simulink model "Horizontal1804"  (R2026b)
settings: Solver=FixedStepDiscrete  StopTime=inf  FixedStep=Official.Step
PostLoadFcn:
  | run(fullfile(fileparts(get_param('StampFly_IMU400','FileName')),'config','startup.m'));
InitFcn:
  | init_imu_flight;
undefined symbols (not defined in the file): Official
libraries: slpidlib x7, simulink x4, mspfiltlib x1
(part 4 of 5)

== system Horizontal1804/FlightControl/TakeoffHoverControl/AttitudeControl/RollAnglePID ==
  Error : Inport
  Dt : Inport  Port=2
  Reset : Inport  Port=3
  Enable : EnablePort
  DedicatedPID : slpidlib/PID Controller  Description=飛行比較用の専用PID。Ideal形式、台形積分・微分フィルター、実測Dt、単精度。  Controller=PID  Form=Ideal  TimeDomain=Discrete-time  UseExternalTs=on  SampleTime=.0025  IntegratorMethod=Trapezoidal  FilterMethod=Trapezoidal  ControllerParametersSource=internal  P=single(5)  I=single(1)/single(4)  UseKiTs=off  D=single(0.039999999105930328)  UseExternalDerivativeSource=off  N=single(1)/(single(0.125)*single(0.039999999105930328))  UseFilter=on  TunerSelectOption=Transfer Function Based (PID Tuner App)  InitialConditionSource=external  InitialConditionForIntegrator=0  InitialConditionForFilter=0  DifferentiatorICPrevScaledInput=0  ExternalReset=level  TrackingMode=off  Kt=1  LimitOutput=off  SatLimitsSource=internal  UpperSaturationLimit=inf  LowerSaturationLimit=-inf  LinearizeAsGain=off  AntiWindupMode=none  Kb=1  LimitIntegrator=on  UpperIntegratorSaturationLimit=single(30000)  LowerIntegratorSaturationLimit=single(-30000)  PGainOutDataTypeStr=single  PProdOutDataTypeStr=single  POutMin=[]  POutMax=[]  IGainOutDataTypeStr=single  IProdOutDataTypeStr=single  IOutMin=[]  IOutMax=[]  DGainOutDataTypeStr=single  DProdOutDataTypeStr=single  DOutMin=[]  DOutMax=[]  NGainOutDataTypeStr=single  NProdOutDataTypeStr=single  NOutMin=[]  NOutMax=[]  SumOutDataTypeStr=single  SumOutMin=[]  SumOutMax=[]  SaturationOutDataTypeStr=single  SaturationOutMin=[]  SaturationOutMax=[]  PParamDataTypeStr=single  PParamMin=[]  PParamMax=[]  IParamDataTypeStr=single  IParamMin=[]  IParamMax=[]  DParamDataTypeStr=single  DParamMin=[]  DParamMax=[]  NParamDataTypeStr=single  NParamMin=[]  NParamMax=[]  KbParamDataTypeStr=single  KbParamMin=[]  KbParamMax=[]  KtParamDataTypeStr=single  KtParamMin=[]  KtParamMax=[]  KbOutDataTypeStr=single  KbOutMin=[]  KbOutMax=[]  KtOutDataTypeStr=single  KtOutMin=[]  KtOutMax=[]  IntegratorOutDataTypeStr=single  IntegratorOutMin=[]  IntegratorOutMax=[]  FilterOutDataTypeStr=single  FilterOutMin=[]  FilterOutMax=[]  SumI1OutDataTypeStr=single  SumI1OutMin=[]  SumI1OutMax=[]  SumI2OutDataTypeStr=single  SumI2OutMin=[]  SumI2OutMax=[]  SumI3OutDataTypeStr=single  SumI3OutMin=[]  SumI3OutMax=[]  SumI4OutDataTypeStr=single  SumI4OutMin=[]  SumI4OutMax=[]  SumDOutDataTypeStr=single  SumDOutMin=[]  SumDOutMax=[]  SumAccumDataTypeStr=single  SumI1AccumDataTypeStr=single  SumI2AccumDataTypeStr=single  SumI3AccumDataTypeStr=single  SumI4AccumDataTypeStr=single  SumDAccumDataTypeStr=single  DifferentiatorOutDataTypeStr=single  DifferentiatorOutMin=[]  DifferentiatorOutMax=[]  FilterDiffOutCoefMin=[]  FilterDiffOutCoefMax=[]  ReciprocalOutDataTypeStr=single  ReciprocalOutMin=[]  ReciprocalOutMax=[]  SumDenOutDataTypeStr=single  SumDenOutMin=[]  SumDenOutMax=[]  SumNumOutDataTypeStr=single  SumNumOutMin=[]  SumNumOutMax=[]  SumDenAccumDataTypeStr=single  SumNumAccumDataTypeStr=single  DivideOutDataTypeStr=single  DivideOutMin=[]  DivideOutMax=[]  UdiffTsProdOutDataTypeStr=single  UdiffTsProdOutMin=[]  UdiffTsProdOutMax=[]  NTsProdOutDataTypeStr=single  NTsProdOutMin=[]  NTsProdOutMax=[]  UintegralTsProdOutDataTypeStr=single  UintegralTsProdOutMin=[]  UintegralTsProdOutMax=[]  UngainTsProdOutDataTypeStr=single  UngainTsProdOutMin=[]  UngainTsProdOutMax=[]  ClampingZeroOutDataTypeStr=single  ClampingZeroOutMin=[]  ClampingZeroOutMax=[]  FilterDenConstantOutDataTypeStr=single  FilterDenConstantOutMin=[]  FilterDenConstantOutMax=[]  PCopyOutDataTypeStr=single  PCopyOutMin=[]  PCopyOutMax=[]  NCopyOutDataTypeStr=single  NCopyOutMin=[]  NCopyOutMax=[]  IntegratorContinuousStateAttributes=''  IntegratorStateMustResolveToSignalObject=off  IntegratorRTWStateStorageClass=Auto  FilterContinuousStateAttributes=''  FilterStateMustResolveToSignalObject=off  FilterRTWStateStorageClass=Auto  ParallelPVariant=Passthrough  IdealPVariant=InternalParameters  IVariant=InternalParameters  DVariant=InternalParameters  IntegratorVariant=Discrete  SatVariant=Disabled  AWVariant=Passthrough  PCopyVariant=Disabled  TRVariant=Disabled  FdbkBlocksVariant=Forward  IdealPFdbkVariant=Disabled  SatFdbkVariant=Disabled  DerivativeFilterVariant=TrapezoidalFilter  NVariant=InternalParameters  NCopyVariant=InternalParameters  FilterICVariant=ExternalICs  IntegratorICVariant=ExternalICs  ExternalResetVariant=ExternalReset  TRSumVariant=Passthrough  SumFdbkVariant=Disabled  SumVariant=Sum_PID  TsampFilterVariant=ExternalTs  TsampNgainVariant=Passthrough  TsampIntegralVariant=ExternalTs  ExternalSaturationOutDataTypeStr=Inherit: Same as second input  DerivativeSourceVariant=ErrorSignal  PreIntVariant=InternalPreInt
      settings: LibrarySourceBlock=simulink/Discrete/Discrete PID Controller
  ZeroInitialCondition : Constant  Description=ZeroInitialCondition：固定値 single(0) を出力します。意味と単位は親の機能説明と信号名を参照します。  Value=single(0)
  Output : Outport
  wires:
  DedicatedPID/1 -> Output/1
  Dt/1 -> DedicatedPID/5
  ZeroInitialCondition/1 -> DedicatedPID/4, DedicatedPID/3
  Reset/1 -> DedicatedPID/2
  Error/1 -> DedicatedPID/1

== system Horizontal1804/FlightControl/TakeoffHoverControl/BodyRateControl/PitchRatePID ==
  Error : Inport
  Dt : Inport  Port=2
  Reset : Inport  Port=3
  Enable : EnablePort
  DedicatedPID : slpidlib/PID Controller  Description=飛行比較用の専用PID。Ideal形式、台形積分・微分フィルター、実測Dt、単精度。  Controller=PID  Form=Ideal  TimeDomain=Discrete-time  UseExternalTs=on  SampleTime=.0025  IntegratorMethod=Trapezoidal  FilterMethod=Trapezoidal  ControllerParametersSource=internal  P=single(0.94999998807907104)  I=single(1)/single(0.69999998807907104)  UseKiTs=off  D=single(0.02500000037252903)  UseExternalDerivativeSource=off  N=single(1)/(single(0.125)*single(0.02500000037252903))  UseFilter=on  TunerSelectOption=Transfer Function Based (PID Tuner App)  InitialConditionSource=external  InitialConditionForIntegrator=0  InitialConditionForFilter=0  DifferentiatorICPrevScaledInput=0  ExternalReset=level  TrackingMode=off  Kt=1  LimitOutput=off  SatLimitsSource=internal  UpperSaturationLimit=inf  LowerSaturationLimit=-inf  LinearizeAsGain=off  AntiWindupMode=none  Kb=1  LimitIntegrator=on  UpperIntegratorSaturationLimit=single(30000)  LowerIntegratorSaturationLimit=single(-30000)  PGainOutDataTypeStr=single  PProdOutDataTypeStr=single  POutMin=[]  POutMax=[]  IGainOutDataTypeStr=single  IProdOutDataTypeStr=single  IOutMin=[]  IOutMax=[]  DGainOutDataTypeStr=single  DProdOutDataTypeStr=single  DOutMin=[]  DOutMax=[]  NGainOutDataTypeStr=single  NProdOutDataTypeStr=single  NOutMin=[]  NOutMax=[]  SumOutDataTypeStr=single  SumOutMin=[]  SumOutMax=[]  SaturationOutDataTypeStr=single  SaturationOutMin=[]  SaturationOutMax=[]  PParamDataTypeStr=single  PParamMin=[]  PParamMax=[]  IParamDataTypeStr=single  IParamMin=[]  IParamMax=[]  DParamDataTypeStr=single  DParamMin=[]  DParamMax=[]  NParamDataTypeStr=single  NParamMin=[]  NParamMax=[]  KbParamDataTypeStr=single  KbParamMin=[]  KbParamMax=[]  KtParamDataTypeStr=single  KtParamMin=[]  KtParamMax=[]  KbOutDataTypeStr=single  KbOutMin=[]  KbOutMax=[]  KtOutDataTypeStr=single  KtOutMin=[]  KtOutMax=[]  IntegratorOutDataTypeStr=single  IntegratorOutMin=[]  IntegratorOutMax=[]  FilterOutDataTypeStr=single  FilterOutMin=[]  FilterOutMax=[]  SumI1OutDataTypeStr=single  SumI1OutMin=[]  SumI1OutMax=[]  SumI2OutDataTypeStr=single  SumI2OutMin=[]  SumI2OutMax=[]  SumI3OutDataTypeStr=single  SumI3OutMin=[]  SumI3OutMax=[]  SumI4OutDataTypeStr=single  SumI4OutMin=[]  SumI4OutMax=[]  SumDOutDataTypeStr=single  SumDOutMin=[]  SumDOutMax=[]  SumAccumDataTypeStr=single  SumI1AccumDataTypeStr=single  SumI2AccumDataTypeStr=single  SumI3AccumDataTypeStr=single  SumI4AccumDataTypeStr=single  SumDAccumDataTypeStr=single  DifferentiatorOutDataTypeStr=single  DifferentiatorOutMin=[]  DifferentiatorOutMax=[]  FilterDiffOutCoefMin=[]  FilterDiffOutCoefMax=[]  ReciprocalOutDataTypeStr=single  ReciprocalOutMin=[]  ReciprocalOutMax=[]  SumDenOutDataTypeStr=single  SumDenOutMin=[]  SumDenOutMax=[]  SumNumOutDataTypeStr=single  SumNumOutMin=[]  SumNumOutMax=[]  SumDenAccumDataTypeStr=single  SumNumAccumDataTypeStr=single  DivideOutDataTypeStr=single  DivideOutMin=[]  DivideOutMax=[]  UdiffTsProdOutDataTypeStr=single  UdiffTsProdOutMin=[]  UdiffTsProdOutMax=[]  NTsProdOutDataTypeStr=single  NTsProdOutMin=[]  NTsProdOutMax=[]  UintegralTsProdOutDataTypeStr=single  UintegralTsProdOutMin=[]  UintegralTsProdOutMax=[]  UngainTsProdOutDataTypeStr=single  UngainTsProdOutMin=[]  UngainTsProdOutMax=[]  ClampingZeroOutDataTypeStr=single  ClampingZeroOutMin=[]  ClampingZeroOutMax=[]  FilterDenConstantOutDataTypeStr=single  FilterDenConstantOutMin=[]  FilterDenConstantOutMax=[]  PCopyOutDataTypeStr=single  PCopyOutMin=[]  PCopyOutMax=[]  NCopyOutDataTypeStr=single  NCopyOutMin=[]  NCopyOutMax=[]  IntegratorContinuousStateAttributes=''  IntegratorStateMustResolveToSignalObject=off  IntegratorRTWStateStorageClass=Auto  FilterContinuousStateAttributes=''  FilterStateMustResolveToSignalObject=off  FilterRTWStateStorageClass=Auto  ParallelPVariant=Passthrough  IdealPVariant=InternalParameters  IVariant=InternalParameters  DVariant=InternalParameters  IntegratorVariant=Discrete  SatVariant=Disabled  AWVariant=Passthrough  PCopyVariant=Disabled  TRVariant=Disabled  FdbkBlocksVariant=Forward  IdealPFdbkVariant=Disabled  SatFdbkVariant=Disabled  DerivativeFilterVariant=TrapezoidalFilter  NVariant=InternalParameters  NCopyVariant=InternalParameters  FilterICVariant=ExternalICs  IntegratorICVariant=ExternalICs  ExternalResetVariant=ExternalReset  TRSumVariant=Passthrough  SumFdbkVariant=Disabled  SumVariant=Sum_PID  TsampFilterVariant=ExternalTs  TsampNgainVariant=Passthrough  TsampIntegralVariant=ExternalTs  ExternalSaturationOutDataTypeStr=Inherit: Same as second input  DerivativeSourceVariant=ErrorSignal  PreIntVariant=InternalPreInt
      settings: LibrarySourceBlock=simulink/Discrete/Discrete PID Controller
  ZeroInitialCondition : Constant  Description=ZeroInitialCondition：固定値 single(0) を出力します。意味と単位は親の機能説明と信号名を参照します。  Value=single(0)
  Output : Outport
  wires:
  DedicatedPID/1 -> Output/1
  Dt/1 -> DedicatedPID/5
  ZeroInitialCondition/1 -> DedicatedPID/4, DedicatedPID/3
  Reset/1 -> DedicatedPID/2
  Error/1 -> DedicatedPID/1

== system Horizontal1804/FlightControl/TakeoffHoverControl/BodyRateControl/RollRatePID ==
  Error : Inport
  Dt : Inport  Port=2
  Reset : Inport  Port=3
  Enable : EnablePort
  DedicatedPID : slpidlib/PID Controller  Description=飛行比較用の専用PID。Ideal形式、台形積分・微分フィルター、実測Dt、単精度。  Controller=PID  Form=Ideal  TimeDomain=Discrete-time  UseExternalTs=on  SampleTime=.0025  IntegratorMethod=Trapezoidal  FilterMethod=Trapezoidal  ControllerParametersSource=internal  P=single(0.64999997615814209)  I=single(1)/single(0.69999998807907104)  UseKiTs=off  D=single(0.0099999997764825821)  UseExternalDerivativeSource=off  N=single(1)/(single(0.125)*single(0.0099999997764825821))  UseFilter=on  TunerSelectOption=Transfer Function Based (PID Tuner App)  InitialConditionSource=external  InitialConditionForIntegrator=0  InitialConditionForFilter=0  DifferentiatorICPrevScaledInput=0  ExternalReset=level  TrackingMode=off  Kt=1  LimitOutput=off  SatLimitsSource=internal  UpperSaturationLimit=inf  LowerSaturationLimit=-inf  LinearizeAsGain=off  AntiWindupMode=none  Kb=1  LimitIntegrator=on  UpperIntegratorSaturationLimit=single(30000)  LowerIntegratorSaturationLimit=single(-30000)  PGainOutDataTypeStr=single  PProdOutDataTypeStr=single  POutMin=[]  POutMax=[]  IGainOutDataTypeStr=single  IProdOutDataTypeStr=single  IOutMin=[]  IOutMax=[]  DGainOutDataTypeStr=single  DProdOutDataTypeStr=single  DOutMin=[]  DOutMax=[]  NGainOutDataTypeStr=single  NProdOutDataTypeStr=single  NOutMin=[]  NOutMax=[]  SumOutDataTypeStr=single  SumOutMin=[]  SumOutMax=[]  SaturationOutDataTypeStr=single  SaturationOutMin=[]  SaturationOutMax=[]  PParamDataTypeStr=single  PParamMin=[]  PParamMax=[]  IParamDataTypeStr=single  IParamMin=[]  IParamMax=[]  DParamDataTypeStr=single  DParamMin=[]  DParamMax=[]  NParamDataTypeStr=single  NParamMin=[]  NParamMax=[]  KbParamDataTypeStr=single  KbParamMin=[]  KbParamMax=[]  KtParamDataTypeStr=single  KtParamMin=[]  KtParamMax=[]  KbOutDataTypeStr=single  KbOutMin=[]  KbOutMax=[]  KtOutDataTypeStr=single  KtOutMin=[]  KtOutMax=[]  IntegratorOutDataTypeStr=single  IntegratorOutMin=[]  IntegratorOutMax=[]  FilterOutDataTypeStr=single  FilterOutMin=[]  FilterOutMax=[]  SumI1OutDataTypeStr=single  SumI1OutMin=[]  SumI1OutMax=[]  SumI2OutDataTypeStr=single  SumI2OutMin=[]  SumI2OutMax=[]  SumI3OutDataTypeStr=single  SumI3OutMin=[]  SumI3OutMax=[]  SumI4OutDataTypeStr=single  SumI4OutMin=[]  SumI4OutMax=[]  SumDOutDataTypeStr=single  SumDOutMin=[]  SumDOutMax=[]  SumAccumDataTypeStr=single  SumI1AccumDataTypeStr=single  SumI2AccumDataTypeStr=single  SumI3AccumDataTypeStr=single  SumI4AccumDataTypeStr=single  SumDAccumDataTypeStr=single  DifferentiatorOutDataTypeStr=single  DifferentiatorOutMin=[]  DifferentiatorOutMax=[]  FilterDiffOutCoefMin=[]  FilterDiffOutCoefMax=[]  ReciprocalOutDataTypeStr=single  ReciprocalOutMin=[]  ReciprocalOutMax=[]  SumDenOutDataTypeStr=single  SumDenOutMin=[]  SumDenOutMax=[]  SumNumOutDataTypeStr=single  SumNumOutMin=[]  SumNumOutMax=[]  SumDenAccumDataTypeStr=single  SumNumAccumDataTypeStr=single  DivideOutDataTypeStr=single  DivideOutMin=[]  DivideOutMax=[]  UdiffTsProdOutDataTypeStr=single  UdiffTsProdOutMin=[]  UdiffTsProdOutMax=[]  NTsProdOutDataTypeStr=single  NTsProdOutMin=[]  NTsProdOutMax=[]  UintegralTsProdOutDataTypeStr=single  UintegralTsProdOutMin=[]  UintegralTsProdOutMax=[]  UngainTsProdOutDataTypeStr=single  UngainTsProdOutMin=[]  UngainTsProdOutMax=[]  ClampingZeroOutDataTypeStr=single  ClampingZeroOutMin=[]  ClampingZeroOutMax=[]  FilterDenConstantOutDataTypeStr=single  FilterDenConstantOutMin=[]  FilterDenConstantOutMax=[]  PCopyOutDataTypeStr=single  PCopyOutMin=[]  PCopyOutMax=[]  NCopyOutDataTypeStr=single  NCopyOutMin=[]  NCopyOutMax=[]  IntegratorContinuousStateAttributes=''  IntegratorStateMustResolveToSignalObject=off  IntegratorRTWStateStorageClass=Auto  FilterContinuousStateAttributes=''  FilterStateMustResolveToSignalObject=off  FilterRTWStateStorageClass=Auto  ParallelPVariant=Passthrough  IdealPVariant=InternalParameters  IVariant=InternalParameters  DVariant=InternalParameters  IntegratorVariant=Discrete  SatVariant=Disabled  AWVariant=Passthrough  PCopyVariant=Disabled  TRVariant=Disabled  FdbkBlocksVariant=Forward  IdealPFdbkVariant=Disabled  SatFdbkVariant=Disabled  DerivativeFilterVariant=TrapezoidalFilter  NVariant=InternalParameters  NCopyVariant=InternalParameters  FilterICVariant=ExternalICs  IntegratorICVariant=ExternalICs  ExternalResetVariant=ExternalReset  TRSumVariant=Passthrough  SumFdbkVariant=Disabled  SumVariant=Sum_PID  TsampFilterVariant=ExternalTs  TsampNgainVariant=Passthrough  TsampIntegralVariant=ExternalTs  ExternalSaturationOutDataTypeStr=Inherit: Same as second input  DerivativeSourceVariant=ErrorSignal  PreIntVariant=InternalPreInt
      settings: LibrarySourceBlock=simulink/Discrete/Discrete PID Controller
  ZeroInitialCondition : Constant  Description=ZeroInitialCondition：固定値 single(0) を出力します。意味と単位は親の機能説明と信号名を参照します。  Value=single(0)
  Output : Outport
  wires:
  DedicatedPID/1 -> Output/1
  Dt/1 -> DedicatedPID/5
  ZeroInitialCondition/1 -> DedicatedPID/3, DedicatedPID/4
  Reset/1 -> DedicatedPID/2
  Error/1 -> DedicatedPID/1

== system Horizontal1804/FlightControl/TakeoffHoverControl/BodyRateControl/YawRatePID ==
  Error : Inport
  Dt : Inport  Port=2
  Reset : Inport  Port=3
  Enable : EnablePort
  DedicatedPID : slpidlib/PID Controller  Description=飛行比較用の専用PID。Ideal形式、台形積分・微分フィルター、実測Dt、単精度。  Controller=PID  Form=Ideal  TimeDomain=Discrete-time  UseExternalTs=on  SampleTime=.0025  IntegratorMethod=Trapezoidal  FilterMethod=Trapezoidal  ControllerParametersSource=internal  P=single(3)  I=single(1)/single(0.80000001192092896)  UseKiTs=off  D=single(0.0099999997764825821)  UseExternalDerivativeSource=off  N=single(1)/(single(0.125)*single(0.0099999997764825821))  UseFilter=on  TunerSelectOption=Transfer Function Based (PID Tuner App)  InitialConditionSource=external  InitialConditionForIntegrator=0  InitialConditionForFilter=0  DifferentiatorICPrevScaledInput=0  ExternalReset=level  TrackingMode=off  Kt=1  LimitOutput=off  SatLimitsSource=internal  UpperSaturationLimit=inf  LowerSaturationLimit=-inf  LinearizeAsGain=off  AntiWindupMode=none  Kb=1  LimitIntegrator=on  UpperIntegratorSaturationLimit=single(30000)  LowerIntegratorSaturationLimit=single(-30000)  PGainOutDataTypeStr=single  PProdOutDataTypeStr=single  POutMin=[]  POutMax=[]  IGainOutDataTypeStr=single  IProdOutDataTypeStr=single  IOutMin=[]  IOutMax=[]  DGainOutDataTypeStr=single  DProdOutDataTypeStr=single  DOutMin=[]  DOutMax=[]  NGainOutDataTypeStr=single  NProdOutDataTypeStr=single  NOutMin=[]  NOutMax=[]  SumOutDataTypeStr=single  SumOutMin=[]  SumOutMax=[]  SaturationOutDataTypeStr=single  SaturationOutMin=[]  SaturationOutMax=[]  PParamDataTypeStr=single  PParamMin=[]  PParamMax=[]  IParamDataTypeStr=single  IParamMin=[]  IParamMax=[]  DParamDataTypeStr=single  DParamMin=[]  DParamMax=[]  NParamDataTypeStr=single  NParamMin=[]  NParamMax=[]  KbParamDataTypeStr=single  KbParamMin=[]  KbParamMax=[]  KtParamDataTypeStr=single  KtParamMin=[]  KtParamMax=[]  KbOutDataTypeStr=single  KbOutMin=[]  KbOutMax=[]  KtOutDataTypeStr=single  KtOutMin=[]  KtOutMax=[]  IntegratorOutDataTypeStr=single  IntegratorOutMin=[]  IntegratorOutMax=[]  FilterOutDataTypeStr=single  FilterOutMin=[]  FilterOutMax=[]  SumI1OutDataTypeStr=single  SumI1OutMin=[]  SumI1OutMax=[]  SumI2OutDataTypeStr=single  SumI2OutMin=[]  SumI2OutMax=[]  SumI3OutDataTypeStr=single  SumI3OutMin=[]  SumI3OutMax=[]  SumI4OutDataTypeStr=single  SumI4OutMin=[]  SumI4OutMax=[]  SumDOutDataTypeStr=single  SumDOutMin=[]  SumDOutMax=[]  SumAccumDataTypeStr=single  SumI1AccumDataTypeStr=single  SumI2AccumDataTypeStr=single  SumI3AccumDataTypeStr=single  SumI4AccumDataTypeStr=single  SumDAccumDataTypeStr=single  DifferentiatorOutDataTypeStr=single  DifferentiatorOutMin=[]  DifferentiatorOutMax=[]  FilterDiffOutCoefMin=[]  FilterDiffOutCoefMax=[]  ReciprocalOutDataTypeStr=single  ReciprocalOutMin=[]  ReciprocalOutMax=[]  SumDenOutDataTypeStr=single  SumDenOutMin=[]  SumDenOutMax=[]  SumNumOutDataTypeStr=single  SumNumOutMin=[]  SumNumOutMax=[]  SumDenAccumDataTypeStr=single  SumNumAccumDataTypeStr=single  DivideOutDataTypeStr=single  DivideOutMin=[]  DivideOutMax=[]  UdiffTsProdOutDataTypeStr=single  UdiffTsProdOutMin=[]  UdiffTsProdOutMax=[]  NTsProdOutDataTypeStr=single  NTsProdOutMin=[]  NTsProdOutMax=[]  UintegralTsProdOutDataTypeStr=single  UintegralTsProdOutMin=[]  UintegralTsProdOutMax=[]  UngainTsProdOutDataTypeStr=single  UngainTsProdOutMin=[]  UngainTsProdOutMax=[]  ClampingZeroOutDataTypeStr=single  ClampingZeroOutMin=[]  ClampingZeroOutMax=[]  FilterDenConstantOutDataTypeStr=single  FilterDenConstantOutMin=[]  FilterDenConstantOutMax=[]  PCopyOutDataTypeStr=single  PCopyOutMin=[]  PCopyOutMax=[]  NCopyOutDataTypeStr=single  NCopyOutMin=[]  NCopyOutMax=[]  IntegratorContinuousStateAttributes=''  IntegratorStateMustResolveToSignalObject=off  IntegratorRTWStateStorageClass=Auto  FilterContinuousStateAttributes=''  FilterStateMustResolveToSignalObject=off  FilterRTWStateStorageClass=Auto  ParallelPVariant=Passthrough  IdealPVariant=InternalParameters  IVariant=InternalParameters  DVariant=InternalParameters  IntegratorVariant=Discrete  SatVariant=Disabled  AWVariant=Passthrough  PCopyVariant=Disabled  TRVariant=Disabled  FdbkBlocksVariant=Forward  IdealPFdbkVariant=Disabled  SatFdbkVariant=Disabled  DerivativeFilterVariant=TrapezoidalFilter  NVariant=InternalParameters  NCopyVariant=InternalParameters  FilterICVariant=ExternalICs  IntegratorICVariant=ExternalICs  ExternalResetVariant=ExternalReset  TRSumVariant=Passthrough  SumFdbkVariant=Disabled  SumVariant=Sum_PID  TsampFilterVariant=ExternalTs  TsampNgainVariant=Passthrough  TsampIntegralVariant=ExternalTs  ExternalSaturationOutDataTypeStr=Inherit: Same as second input  DerivativeSourceVariant=ErrorSignal  PreIntVariant=InternalPreInt
      settings: LibrarySourceBlock=simulink/Discrete/Discrete PID Controller
  ZeroInitialCondition : Constant  Description=ZeroInitialCondition：固定値 single(0) を出力します。意味と単位は親の機能説明と信号名を参照します。  Value=single(0)
  Output : Outport
  wires:
  DedicatedPID/1 -> Output/1
  Dt/1 -> DedicatedPID/5
  ZeroInitialCondition/1 -> DedicatedPID/3, DedicatedPID/4
  Reset/1 -> DedicatedPID/2
  Error/1 -> DedicatedPID/1

== system Horizontal1804/FlightControl/TakeoffHoverControl/FlightCommand/ControlGating ==
  CommandMode : Inport
  ModeContext : Inport  Port=2
  ThrustState : Inport  Port=3
  CommandModeFields : BusSelector  Description=CommandModeFields：バスから RawThrust,ManualAltitude,AltitudeEnabled,ControlMode を選びます。元のベクトルの成分順序は変更しません。  OutputSignals=RawThrust,ManualAltitude,AltitudeEnabled,ControlMode
  ControlContextBus : BusCreator  Description=ControlContextBus：異なる単位・型を持つ関連信号を名前付きバスにまとめます。入力線の信号名が項目名です。  Inputs=5
  ControlEnableReset : MATLAB Function  Description=共通推力指令の平滑化と各 PID の実行・リセット条件を決めます。推力を 3.7 V 基準の Duty に換算し、0.1 未満なら PID をリセットします。高度・角度・速度ループは操縦モードに応じて個別に有効にします。  TreatAsAtomicUnit=on
  ModeContextFields : BusSelector  Description=ModeContextFields：バスから FlightContext.Branch,Dt,Mode を選びます。元のベクトルの成分順序は変更しません。  OutputSignals=FlightContext.Branch,Dt,Mode
  ThrustStateFields : BusSelector  Description=ThrustStateFields：バスから FilteredThrust,HeldThrust を選びます。元のベクトルの成分順序は変更しません。  OutputSignals=FilteredThrust,HeldThrust
  ThrustRequest : Outport
  ControlContext : Outport  Port=2
  wires:
  ThrustState/1 -> ThrustStateFields/1
  ModeContext/1 -> ModeContextFields/1
  CommandMode/1 -> CommandModeFields/1
  CommandModeFields/1 -> ControlEnableReset/1(arg_arg_raw)  "<RawThrust>"
  CommandModeFields/2 -> ControlEnableReset/2(arg_arg_manual)  "<ManualAltitude>"
  CommandModeFields/3 -> ControlEnableReset/3(arg_arg_auto)  "<AltitudeEnabled>"
  ModeContextFields/1 -> ControlEnableReset/4(arg_branch)  "<Branch>"
  ModeContextFields/2 -> ControlEnableReset/6(arg_arg_dt)  "<Dt>"
  CommandModeFields/4 -> ControlEnableReset/5(arg_arg_controlMode)  "<ControlMode>"
  ModeContextFields/3 -> ControlEnableReset/9(arg_arg_mode)  "<Mode>"
  ThrustStateFields/1 -> ControlEnableReset/7(arg_arg_oldFilter)  "<FilteredThrust>"
  ThrustStateFields/2 -> ControlEnableReset/8(arg_arg_lastThrust)  "<HeldThrust>"
  ControlEnableReset/1(arg_arg_command) -> ThrustRequest/1  "ThrustRequest"
  ControlEnableReset/2(arg_arg_run) -> ControlContextBus/1  "Run"
  ControlEnableReset/3(arg_arg_reset) -> ControlContextBus/2  "Reset"
  ControlEnableReset/4(arg_arg_altEnable) -> ControlContextBus/3  "AltitudeEnabled"
  ControlEnableReset/5(arg_arg_angleEnable) -> ControlContextBus/4  "AngleEnabled"
  ControlEnableReset/6(arg_arg_velEnable) -> ControlContextBus/5  "VelocityEnabled"
  ControlContextBus/1 -> ControlContext/1  "ControlContext"

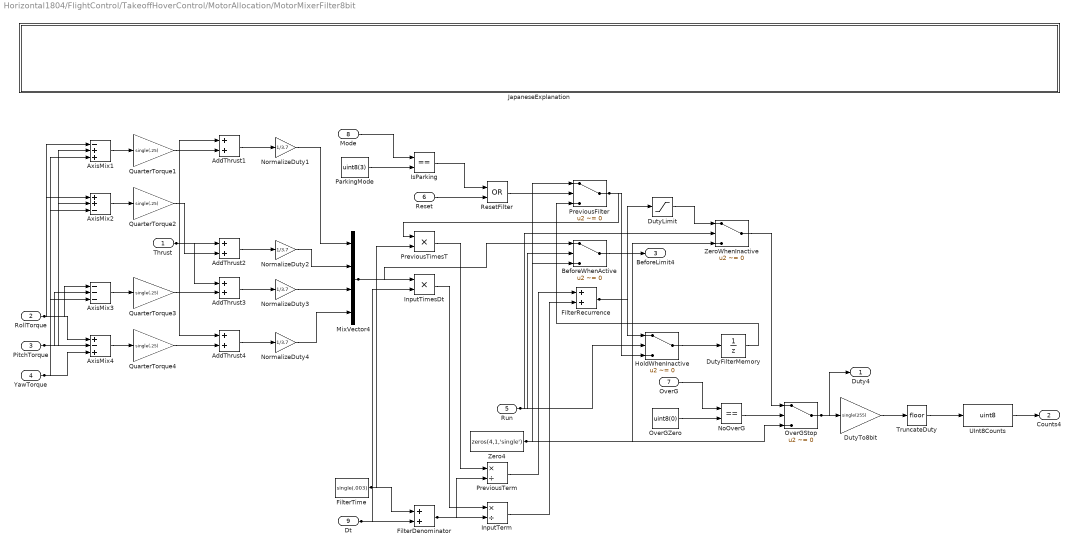
== system Horizontal1804/FlightControl/TakeoffHoverControl/MotorAllocation/MotorMixerFilter8bit ==
  Thrust : Inport
  RollTorque : Inport  Port=2
  PitchTorque : Inport  Port=3
  YawTorque : Inport  Port=4
  Run : Inport  Port=5
  Reset : Inport  Port=6
  OverG : Inport  Port=7
  Mode : Inport  Port=8
  Dt : Inport  Port=9
  AddThrust1 : Sum  Description=AddThrust1：入力を ++ の符号で加減算します。ベクトルでは各成分に同じ演算を適用します。
  AddThrust2 : Sum  Description=AddThrust2：入力を ++ の符号で加減算します。ベクトルでは各成分に同じ演算を適用します。
  AddThrust3 : Sum  Description=AddThrust3：入力を ++ の符号で加減算します。ベクトルでは各成分に同じ演算を適用します。
  AddThrust4 : Sum  Description=AddThrust4：入力を ++ の符号で加減算します。ベクトルでは各成分に同じ演算を適用します。
  AxisMix1 : Sum  Description=AxisMix1：入力を -++ の符号で加減算します。ベクトルでは各成分に同じ演算を適用します。  Inputs=-++
  AxisMix2 : Sum  Description=AxisMix2：入力を ++- の符号で加減算します。ベクトルでは各成分に同じ演算を適用します。  Inputs=++-
  AxisMix3 : Sum  Description=AxisMix3：入力を --- の符号で加減算します。ベクトルでは各成分に同じ演算を適用します。  Inputs=---
  AxisMix4 : Sum  Description=AxisMix4：入力を +-+ の符号で加減算します。ベクトルでは各成分に同じ演算を適用します。  Inputs=+-+
  BeforeWhenActive : Switch  Description=BeforeWhenActive：条件入力で更新値と保持・リセット値を選びます。条件は u2 ~= 0。  Criteria=u2 ~= 0  SaturateOnIntegerOverflow=off  InputSameDT=off
  DutyFilterMemory : UnitDelay  Description=DutyFilterMemory：前周期の値を保持して出力します。更新順序と状態保持に必要な 1 周期遅延です。初期値 zeros(4,1,'single')、周期 Official.Step 秒。  InitialCondition=zeros(4,1,'single')  SampleTime=Official.Step
  DutyLimit : Saturate  Description=DutyLimit：下限 single(0)、上限 single(.95) で入力を制限します。  UpperLimit=single(.95)  LowerLimit=single(0)
  DutyTo8bit : Gain  Description=DutyTo8bit：入力に single(255) を掛けます。座標変換・単位換算・制御係数は用途ごとに維持します。  Gain=single(255)
  FilterDenominator : Sum  Description=FilterDenominator：入力を ++ の符号で加減算します。ベクトルでは各成分に同じ演算を適用します。
  FilterRecurrence : Sum  Description=FilterRecurrence：入力を ++ の符号で加減算します。ベクトルでは各成分に同じ演算を適用します。
  FilterTime : Constant  Description=FilterTime：固定値 single(.003) を出力します。意味と単位は親の機能説明と信号名を参照します。  Value=single(.003)
  HoldWhenInactive : Switch  Description=HoldWhenInactive：条件入力で更新値と保持・リセット値を選びます。条件は u2 ~= 0。  Criteria=u2 ~= 0  SaturateOnIntegerOverflow=off  InputSameDT=off
  InputTerm : Product  Description=InputTerm：入力の乗算・除算（*/）を行います。フィルターは既存の演算順序を保ちます。  Inputs=*/
  InputTimesDt : Product  Description=InputTimesDt：入力の乗算・除算（2）を行います。フィルターは既存の演算順序を保ちます。
  IsParking : RelationalOperator  Operator===  OutDataTypeStr=boolean  RndMeth=Simplest  InputSameDT=off
  JapaneseExplanation : Subsystem  Description=4 モーターの符号付き配分、平滑化、飽和、8 bit 変換を一連の処理として示します。モーター順 [FR, FL, RR, RL] は出力・ログでも同じです。
      mask help: 4 モーターの符号付き配分、平滑化、飽和、8 bit 変換を一連の処理として示します。モーター順 [FR, FL, RR, RL] は出力・ログでも同じです。
      mask Display: disp(sprintf('4 モーターの符号付き配分、平滑化、飽和、8 bit 変換を一連の処理として示します。\nモーター順 [FR, FL, RR, RL] は出力・ログでも同じです。'));
  MixVector4 : Mux  Description=MixVector4：同じ型の値を入力端子の順でベクトルに結合します。ログ仕様・モーター順に対応する結合は順序を保ちます。
  NoOverG : RelationalOperator  Operator===  OutDataTypeStr=boolean  RndMeth=Simplest  InputSameDT=off
  NormalizeDuty1 : Gain  Description=NormalizeDuty1：入力に 1/3.7 を掛けます。座標変換・単位換算・制御係数は用途ごとに維持します。  Gain=1/3.7  OutDataTypeStr=single
  NormalizeDuty2 : Gain  Description=NormalizeDuty2：入力に 1/3.7 を掛けます。座標変換・単位換算・制御係数は用途ごとに維持します。  Gain=1/3.7  OutDataTypeStr=single
  NormalizeDuty3 : Gain  Description=NormalizeDuty3：入力に 1/3.7 を掛けます。座標変換・単位換算・制御係数は用途ごとに維持します。  Gain=1/3.7  OutDataTypeStr=single
  NormalizeDuty4 : Gain  Description=NormalizeDuty4：入力に 1/3.7 を掛けます。座標変換・単位換算・制御係数は用途ごとに維持します。  Gain=1/3.7  OutDataTypeStr=single
  OverGStop : Switch  Description=OverGStop：条件入力で更新値と保持・リセット値を選びます。条件は u2 ~= 0。  Criteria=u2 ~= 0  SaturateOnIntegerOverflow=off  InputSameDT=off
  OverGZero : Constant  Description=OverGZero：固定値 uint8(0) を出力します。意味と単位は親の機能説明と信号名を参照します。  Value=uint8(0)
  ParkingMode : Constant  Description=ParkingMode：固定値 uint8(3) を出力します。意味と単位は親の機能説明と信号名を参照します。  Value=uint8(3)
  PreviousFilter : Switch  Description=PreviousFilter：条件入力で更新値と保持・リセット値を選びます。条件は u2 ~= 0。  Criteria=u2 ~= 0  SaturateOnIntegerOverflow=off  InputSameDT=off
  PreviousTerm : Product  Description=PreviousTerm：入力の乗算・除算（*/）を行います。フィルターは既存の演算順序を保ちます。  Inputs=*/
  PreviousTimesT : Product  Description=PreviousTimesT：入力の乗算・除算（2）を行います。フィルターは既存の演算順序を保ちます。
  QuarterTorque1 : Gain  Description=QuarterTorque1：入力に single(.25) を掛けます。座標変換・単位換算・制御係数は用途ごとに維持します。  Gain=single(.25)
  QuarterTorque2 : Gain  Description=QuarterTorque2：入力に single(.25) を掛けます。座標変換・単位換算・制御係数は用途ごとに維持します。  Gain=single(.25)
  QuarterTorque3 : Gain  Description=QuarterTorque3：入力に single(.25) を掛けます。座標変換・単位換算・制御係数は用途ごとに維持します。  Gain=single(.25)
  QuarterTorque4 : Gain  Description=QuarterTorque4：入力に single(.25) を掛けます。座標変換・単位換算・制御係数は用途ごとに維持します。  Gain=single(.25)
  ResetFilter : Logic  Operator=OR  AllPortsSameDT=off  OutDataTypeStr=boolean
  TruncateDuty : Rounding
  UInt8Counts : DataTypeConversion  Description=UInt8Counts：後段のバス・演算に合わせて uint8 型へ変換します。  OutDataTypeStr=uint8  SaturateOnIntegerOverflow=off  RndMeth=Floor
  Zero4 : Constant  Description=Zero4：固定値 zeros(4,1,'single') を出力します。意味と単位は親の機能説明と信号名を参照します。  Value=zeros(4,1,'single')
  ZeroWhenInactive : Switch  Description=ZeroWhenInactive：条件入力で更新値と保持・リセット値を選びます。条件は u2 ~= 0。  Criteria=u2 ~= 0  SaturateOnIntegerOverflow=off  InputSameDT=off
  Duty4 : Outport
  Counts4 : Outport  Port=2
  BeforeLimit4 : Outport  Port=3
  wires:
  YawTorque/1 -> AxisMix2/3, AxisMix3/3, AxisMix4/3, AxisMix1/3
  RollTorque/1 -> AxisMix1/1, AxisMix4/1, AxisMix3/1, AxisMix2/1
  PitchTorque/1 -> AxisMix4/2, AxisMix3/2, AxisMix2/2, AxisMix1/2
  MixVector4/1 -> BeforeWhenActive/1, InputTimesDt/1
  AxisMix1/1 -> QuarterTorque1/1
  QuarterTorque1/1 -> AddThrust1/2
  AxisMix2/1 -> QuarterTorque2/1
  NormalizeDuty2/1 -> MixVector4/2
  AxisMix3/1 -> QuarterTorque3/1
  QuarterTorque3/1 -> AddThrust3/2
  AxisMix4/1 -> QuarterTorque4/1
  QuarterTorque2/1 -> AddThrust2/2
  Thrust/1 -> AddThrust1/1, AddThrust2/1, AddThrust4/1, AddThrust3/1
  QuarterTorque4/1 -> AddThrust4/2
  AddThrust1/1 -> NormalizeDuty1/1
  TruncateDuty/1 -> UInt8Counts/1
  AddThrust2/1 -> NormalizeDuty2/1
  DutyFilterMemory/1 -> PreviousFilter/3
  AddThrust3/1 -> NormalizeDuty3/1
  AddThrust4/1 -> NormalizeDuty4/1
  NormalizeDuty1/1 -> MixVector4/1
  HoldWhenInactive/1 -> DutyFilterMemory/1
  NormalizeDuty3/1 -> MixVector4/3
  NormalizeDuty4/1 -> MixVector4/4
  Mode/1 -> IsParking/1
  IsParking/1 -> ResetFilter/1
  ParkingMode/1 -> IsParking/2
  FilterTime/1 -> FilterDenominator/1, PreviousTimesT/2
  Dt/1 -> InputTimesDt/2, FilterDenominator/2
  Reset/1 -> ResetFilter/2
  FilterRecurrence/1 -> DutyLimit/1, HoldWhenInactive/1
  PreviousTimesT/1 -> PreviousTerm/1
  OverGStop/1 -> DutyTo8bit/1, Duty4/1
  BeforeWhenActive/1 -> BeforeLimit4/1
  InputTimesDt/1 -> InputTerm/1
  PreviousTerm/1 -> FilterRecurrence/1
  FilterDenominator/1 -> PreviousTerm/2, InputTerm/2
  ResetFilter/1 -> PreviousFilter/2
  Run/1 -> ZeroWhenInactive/2, HoldWhenInactive/2, BeforeWhenActive/2
  Zero4/1 -> OverGStop/3, PreviousFilter/1, BeforeWhenActive/3, ZeroWhenInactive/3
  InputTerm/1 -> FilterRecurrence/2
  DutyTo8bit/1 -> TruncateDuty/1
  PreviousFilter/1 -> PreviousTimesT/1, HoldWhenInactive/3
  DutyLimit/1 -> ZeroWhenInactive/1
  OverG/1 -> NoOverG/1
  OverGZero/1 -> NoOverG/2
  ZeroWhenInactive/1 -> OverGStop/1
  NoOverG/1 -> OverGStop/2
  UInt8Counts/1 -> Counts4/1

== system Horizontal1804/FlightControl/TakeoffHoverControl/MotorAllocation/MotorMixerFilter8bit/JapaneseExplanation ==

== matlab function Horizontal1804/AttitudeAltitudeEstimation/IMUAttitude/FilterInputs ==
  data: rates input; accelMps2 output; accelG input; mode input; reset input; gyroRps output; run output; filterReset output
function [accelMps2,gyroRps,run,filterReset]=IMUFilterInputs(rates,accelG,mode,reset)
% 概要：IMU Filter の入力を準備します。機体座標 XYZ の角速度 [rad/s] と加速度 [g] を、推定器の座標と SI 単位へ変換します。校正中のリセット要求は、推定を再開するまで保持します。
%#codegen
% 1. 入力座標を [Y, X, -Z] に変換し、加速度を m/s² に換算します。静止時に推定器の Z が +g になる NED の定義です。
accelMps2=single([accelG(2),accelG(1),-accelG(3)])*single(9.80665);
gyroRps=single([rates(2),rates(1),-rates(3)]);
% 2. 起動・校正中（Mode 0, 1）は推定を停止し、Mode 2 以降で更新します。
run=mode>uint8(1);
% 3. 停止中には Resettable subsystem も実行されないため、要求を記憶して再開時の最初の更新に渡します。
persistent pendingReset
if isempty(pendingReset),pendingReset=false;end
if reset,pendingReset=true;end
filterReset=pendingReset;
if run,pendingReset=false;end
end

== matlab function Horizontal1804/AttitudeAltitudeEstimation/IMUAttitude/FlightOutputs ==
  data: orientation input; angles output; angularVelocity input; run input; reset input; rawRates input; q output; rates output
function [angles,q,rates]=IMUFlightOutputs(orientation,angularVelocity,run,reset,rawRates)
% 概要：IMU Filter の姿勢とバイアス補正済み角速度を、従来の飛行制御の座標・順序へ戻します。出力は角度 [Roll, Pitch, Yaw] [rad]、クォータニオン [w, x, y, z]、機体 XYZ 角速度 [rad/s] です。
%#codegen
% 1. 推定停止中に公開する前回の角度・姿勢・バイアスを保持します。初期姿勢は単位クォータニオンです。
persistent heldAngles heldQuaternion heldBias
if isempty(heldAngles)
    heldAngles=zeros(3,1,'single');
    heldQuaternion=single([1;0;0;0]);
    heldBias=zeros(3,1,'single');
end
% 2. リセットでは姿勢と角速度バイアスを初期化します。角度は次の推定更新まで前回値を保ちます。
if reset
    heldQuaternion=single([1;0;0;0]);
    heldBias=zeros(3,1,'single');
end
% 3. 補正済み角速度を機体 XYZ に戻し、更新時はその値を PID へ渡します。
correctedRates=single([angularVelocity(2);angularVelocity(1);-angularVelocity(3)]);
% 4. クォータニオンから角度を計算します。asin の入力制限、従来の rad/deg 換算係数、Yaw の 180° オフセットを維持します。
if run
    heldQuaternion=single(orientation(:));
    w=heldQuaternion(1);x=heldQuaternion(2);y=heldQuaternion(3);z=heldQuaternion(4);
    roll=atan2(single(2)*(w*x+y*z),single(1)-single(2)*(x*x+y*y));
    pitch=asin(min(single(1),max(single(-1),single(2)*(w*y-z*x))));
    yaw=atan2(single(2)*(x*y+w*z),single(1)-single(2)*(y*y+z*z));
    heldAngles=[pitch*single(57.29578);roll*single(57.29578); ...
        -(yaw*single(57.29578)+single(180))]*single(pi/180);
    heldBias=single(rawRates(:))-correctedRates;
end
% 5. 出力を公開します。停止中は生のフィルター済み角速度から最後のバイアスを引き、追加の周期遅れを入れません。
angles=heldAngles;q=heldQuaternion;
rates=single(rawRates(:))-heldBias;
if run,rates=correctedRates;end
end

== stateflow chart Horizontal1804/FlightControl/TakeoffHoverControl/FlightCommand/TakeoffLandingCommand ==
  settings: description=|
      | 離陸・ホバリング・着陸の指令生成（400 Hz）
      | Parking: 高度0.5 m/推力0へ初期化。自動離陸: 0〜499周期は3.8 V基準、500〜999周期は実電圧トリム。
      | AutoHover: 1000周期後の基準推力。目標高度0.05〜1.8 m、スティックで更新。
      | ManualAltitude/AutoHover/Landingの遷移条件は図に表示。演算順・状態保持・AltFlag保持は公式互換。
      | Chart内にMATLAB関数は置かない。
  state CommandPhases [parallel]
    settings: executionOrder=1
    state Parking
      en: Base=single(0);Alt=single(.5);Counter=uint16(0);landingActive=false;AltFlag=false;
    state TakeoffReference
      en: ControlMode=uint8(stick(5));AltFlag=true;
      Base=min(single(Counter)/single(1000),(-single(.2448)*single(3.8)+single(1.5892)));Counter=Counter+uint16(1);
      th=stick(4);if th>-.2 && th<.2,th=single(0);end
      Alt=min(max(single(double(Alt)+double(th)*.001),single(.05)),single(1.8));
      if rangeFlag>RangeOld || rangeFlag==20,Base=Base-single(.02);RangeOld=rangeFlag;end
      raw=single(double(Base)*3.7);
    state ManualAltitude
      en: ControlMode=uint8(stick(5));manual=true;th=min(max(stick(4),single(0)),single(1));
      if th>-.2 && th<.2,th=single(0);end
      raw=single((.00413+double(single(3.3)*th-single(5.44)*th*th+single(3.13)*th*th*th))*3.7);
    state TakeoffBattery
      en: ControlMode=uint8(stick(5));AltFlag=true;
      Base=min(single(Counter)/single(1000),(-single(.2448)*voltage+single(1.5892)));Counter=Counter+uint16(1);
      th=stick(4);if th>-.2 && th<.2,th=single(0);end
      Alt=min(max(single(double(Alt)+double(th)*.001),single(.05)),single(1.8));
      if rangeFlag>RangeOld || rangeFlag==20,Base=Base-single(.02);RangeOld=rangeFlag;end
      raw=single(double(Base)*3.7);
    state AutoHover
      en: ControlMode=uint8(stick(5));AltFlag=true;
      Base=(-single(.2448)*voltage+single(1.5892));
      th=stick(4);if th>-.2 && th<.2,th=single(0);end
      Alt=min(max(single(double(Alt)+double(th)*.001),single(.05)),single(1.8));
      if rangeFlag>RangeOld || rangeFlag==20,Base=Base-single(.02);RangeOld=rangeFlag;end
      raw=single(double(Base)*3.7);
    state Landing
      en: AltFlag=false;
      if ~landingActive,landingActive=true;History(:)=height;Base=(-single(.2448)*voltage+single(1.5892));end
      if History(10)>=height,Base=single(double(Base)*.9999);end
      if height<.15,Base=single(double(Base)*.999);end
      if height<.1,landingActive=false;end
      for j=2:10,History(j)=History(j-1);end
      History(1)=height;
    state Hold
    CommandPhases -> (junction 50) : step
    (junction 50) -> AutoHover [order 6] : [mode==2 && uint8(stick(6))==4]
    (junction 50) -> Hold [order 7]
    (junction 50) -> Parking [order 1] : [mode==3]
    (junction 50) -> Landing [order 2] : [mode==5]
    (junction 50) -> TakeoffBattery [order 5] : [mode==2 && uint8(stick(6))==4 && Counter<1000]
    (junction 50) -> TakeoffReference [order 4] : [mode==2 && uint8(stick(6))==4 && Counter<500]
    (default) -> Hold : /{Alt=single(.5);Base=single(0);Counter=uint16(0);RangeOld=uint8(0);landingActive=false;History=zeros(10,1,'single');AltFlag=false;ControlMode=uint8(0);th=single(0);j=double(0);}
    (junction 50) -> ManualAltitude [order 3] : [mode==2 && uint8(stick(6))~=4]
  state CycleOutputs [parallel]
    en: raw=single(0);manual=false;
    send(step,CommandPhases);
    alt=Alt;base=Base;counter=Counter;auto=AltFlag;controlMode=single(ControlMode);
    du: raw=single(0);manual=false;
    send(step,CommandPhases);
    alt=Alt;base=Base;counter=Counter;auto=AltFlag;controlMode=single(ControlMode);
    settings: executionOrder=2
  note: 離陸・ホバリング・着陸の指令生成（400 Hz）
      | Parking: 高度0.5 m/推力0へ初期化。自動離陸: 0〜499周期は3.8 V基準、500〜999周期は実電圧トリム。
      | AutoHover: 1000周期後の基準推力。目標高度0.05〜1.8 m、スティックで更新。
      | ManualAltitude/AutoHover/Landingの遷移条件は図に表示。演算順・状態保持・AltFlag保持は公式互換。
      | Chart内にMATLAB関数は置かない。
  data: stick input single; height input single; voltage input single; rangeFlag input uint8; mode input uint8; alt output single; base output single; counter output uint16; raw output single; auto output boolean; manual output boolean; controlMode output single; Alt local single; Base local single; Counter local uint16; RangeOld local uint8; landingActive local boolean; History local single; AltFlag local boolean; ControlMode local uint8; th local single; j local double
  events: step local FUNCTION_CALL_EVENT

== matlab function Horizontal1804/LEDAndBuzzer/StatusIndicators ==
  data: arg_mode input uint8; arg_color1 output uint32; arg_controlMode input single; arg_altFlag input uint8; arg_lowVoltage input uint8; arg_rcError input uint8; arg_ahrsFlag input uint8; arg_button input uint8; arg_color2 output uint32; arg_tone output uint32; arg_restart output boolean
function [arg_color1,arg_color2,arg_tone,arg_restart]=stepFn(arg_mode,arg_controlMode,arg_altFlag,arg_lowVoltage,arg_rcError,arg_ahrsFlag,arg_button)
% 概要：飛行モード・電池・通信状態を LED 色とブザーへ変換します。待ち時間は 400 Hz のカウンターで管理し、機体ボタンの押下・解放を確認して再起動要求を出します。実際の LED・音・再起動は後段の I/O が行います。
%#codegen
% 1. 点滅、色、起動音、ボタン判定の状態を保持します。
persistent Blink Rainbow C1 C2 Tick AHRSPrev ToneTicks ButtonCount WasPressed;
if isempty(Blink)
 Blink=uint16(0);Rainbow=uint32(255);C1=uint32(0);C2=uint32(0);Tick=uint16(0);AHRSPrev=uint8(0);ToneTicks=uint16(0);ButtonCount=uint8(0);WasPressed=false;
end
% 2. 校正・着陸・飛行・待機の色を選び、低電圧や通信異常の表示を重ねます。
if arg_mode==1,C1=uint32(hex2dec('FF00FF'));C2=C1;
elseif arg_mode==5,C1=uint32(hex2dec('00FF00'));C2=C1;
elseif arg_mode==2
 c=uint32(hex2dec('FFFF00'));
 if arg_controlMode~=0,c=uint32(hex2dec('DC669B'));end
 if arg_altFlag>=1,c=uint32(hex2dec('331155'));end
 if arg_rcError==1,c=uint32(hex2dec('FF0000'));end
 C1=c;C2=c;if arg_lowVoltage>=100,C1=uint32(hex2dec('18EBF9'));end
elseif arg_mode==3
 if arg_lowVoltage<100
  if Blink==0
   top=bitand(Rainbow,uint32(hex2dec('800000')))~=0;Rainbow=bitshift(Rainbow,1);if top,Rainbow=bitor(Rainbow,uint32(1));end
   C1=Rainbow;C2=Rainbow;Blink=Blink+uint16(1);
  end
  Blink=Blink+uint16(1);if Blink>20,Blink=uint16(0);end
 else
  if Blink<10,C1=uint32(hex2dec('18EBF9'));C2=C1;
  elseif Blink<200,C1=uint32(0);C2=uint32(0);else,Blink=uint16(0);end
  Blink=Blink+uint16(1);
 end
 if arg_ahrsFlag~=AHRSPrev && arg_ahrsFlag==1,ToneTicks=uint16(80);end
 AHRSPrev=arg_ahrsFlag;
end
% 3. 起動時は 80 周期（200 ms）ずつ 4 音を鳴らし、その後は要求時だけブザーを出します。
arg_tone=uint32(0);
if Tick<320
 notes=uint32([294 441 350 393]);idx=min(floor(double(Tick)/80)+1,4);arg_tone=notes(idx);Tick=Tick+uint16(1);
elseif ToneTicks>0,arg_tone=uint32(4000);ToneTicks=ToneTicks-uint16(1);end
% 4. 機体ボタンが 4 周期以上押されたことを確認し、解放時に再起動を要求します。
arg_restart=false;
if arg_button==1,ButtonCount=min(ButtonCount+uint8(1),uint8(40));if ButtonCount>=4,WasPressed=true;end
elseif WasPressed,arg_restart=true;WasPressed=false;ButtonCount=uint8(0);else,ButtonCount=uint8(0);end
% 5. 表示用の RGB を輝度 15 相当に縮小します。
arg_color1=scale(C1);arg_color2=scale(C2);
end
% 6. 局所関数：RGB 各成分を取り出して輝度を換算し、24 bit の色へ戻します。
function c=scale(x)
r=bitand(bitshift(x,-16),uint32(255));g=bitand(bitshift(x,-8),uint32(255));b=bitand(x,uint32(255));
c=bitor(bitor(bitshift(uint32(double(r)*15/255),16),bitshift(uint32(double(g)*15/255),8)),uint32(double(b)*15/255));
end

== matlab function Horizontal1804/FlightControl/TakeoffHoverControl/AltitudeControl/SelectVerticalReference ==
  data: arg_zRef input single; arg_vRef output single; arg_mode input uint8; arg_auto input boolean
function arg_vRef=stepFn(arg_zRef,arg_mode,arg_auto)
% 概要：鉛直速度目標を選びます。Auto Altitude 時は高度 PID の目標を使い、手動高度で着陸中（Mode 5）のときだけ -0.15 の降下目標に切り替えます。
%#codegen
% 1. Auto 高度制御を優先する既存の判定順序を保ち、目標を選択します。
arg_vRef=arg_zRef;if ~arg_auto && arg_mode==5,arg_vRef=single(-.15);end
end

== matlab function Horizontal1804/JoystickFeedback40/OfficialTelemetryValues ==
  data: arg_t input single; arg_values output single; arg_dt input single; arg_a input single; arg_r input single; arg_cd input single; arg_accel input single; arg_voltage input single; arg_duty input single; arg_z input single; arg_sd input single; arg_v input single
function arg_values=stepFn(arg_t,arg_dt,arg_a,arg_r,arg_cd,arg_accel,arg_voltage,arg_duty,arg_z,arg_sd,arg_v)
% 概要：JoyStick へ返す公式 120 byte テレメトリの 27 個の float 値を作ります。時刻・姿勢・目標・電池・加速度・速度・高度などを公式の単位と順序へ変換します。送信は後段の専用 I/O ブロックが行います。
%#codegen
% 1. 時刻と dt、姿勢角・角速度を配置します。角度は rad から deg へ変換します。
arg_values=zeros(27,1,'single');arg_values(1:2)=[arg_t;arg_dt];arg_values(3:8)=[arg_a;arg_r]*single(180/pi);
% 2. 制御目標と推力、電圧を配置します。
arg_values(9:13)=arg_cd(6:10)*single(180/pi);arg_values(14)=single(double(arg_cd(5))/3.7);
% 3. 加速度を公式のセンサー軸順と g 単位へ戻します。これは通信形式の変換です。
arg_values(15)=arg_voltage;arg_values(16:18)=arg_accel([2 1 3])/single(9.80665);arg_values(18)=-arg_values(18);
% 4. 鉛直速度、目標、モーター、高度、推定診断を既存の通信順序へ配置します。
arg_values(19:20)=[arg_v;arg_cd(4)];arg_values(21:22)=arg_duty(2:3);
arg_values(23:27)=[arg_cd(1);arg_z;arg_sd(3);arg_sd(1:2)];
end

== matlab function Horizontal1804/FlightControl/TakeoffHoverControl/AltitudeControl/ThrustCorrectionLimits ==
  data: arg_arg_command input single; arg_arg_thrust output single; arg_arg_correction input single; arg_arg_base input single; arg_arg_auto input boolean; arg_arg_manual input boolean; arg_arg_velEnable input boolean; arg_branch input uint8; arg_arg_dt input single; arg_arg_oldFilter input single; arg_arg_lastThrust input single; arg_arg_filter output single; arg_arg_last output single
function [arg_arg_thrust,arg_arg_filter,arg_arg_last]=stepFn(arg_arg_command,arg_arg_correction,arg_arg_base,arg_arg_auto,arg_arg_manual,arg_arg_velEnable,arg_branch,arg_arg_dt,arg_arg_oldFilter,arg_arg_lastThrust)
% 概要：共通推力を決めます。鉛直速度 PID の補正を基準推力へ加え、10 ms で平滑化します。Auto Altitude 時は基準の 0.85～1.15 倍に制限し、指定された分岐では前回推力を保持します。
%#codegen
% 1. 入力推力と前回のフィルター値を準備し、待機・手動の状態を反映します。
arg_arg_thrust=arg_arg_command;arg_arg_filter=arg_arg_oldFilter;
if arg_branch==3,arg_arg_filter=single(0);elseif arg_arg_manual,arg_arg_filter=arg_arg_command;end
% 2. 鉛直速度制御が有効なら、基準＋PID 補正を既存の 3.7 V 基準の推力表現へ換算して平滑化します。
if arg_arg_velEnable
 arg_arg_filter=filterStep(single(double(arg_arg_base+arg_arg_correction)*3.7),arg_arg_dt,single(.01),arg_arg_filter);arg_arg_thrust=arg_arg_filter;
% 3. Auto Altitude の上限・下限を適用します。演算の single/double 変換順も維持します。
 if arg_arg_auto
  if double(arg_arg_thrust)/3.7>double(single(arg_arg_base*single(1.15))),arg_arg_thrust=single(3.7*double(arg_arg_base)*double(single(1.15)));end
  if double(arg_arg_thrust)/3.7<double(single(arg_arg_base*single(.85))),arg_arg_thrust=single(3.7*double(arg_arg_base)*double(single(.85)));end
 end
end
% 4. 前回推力の保持または更新を行い、次周期へ渡します。
if arg_branch==3,arg_arg_thrust=arg_arg_lastThrust;arg_arg_last=arg_arg_lastThrust;else,arg_arg_last=arg_arg_thrust;end
end
% 5. 局所関数：前回値と入力値の一次低域フィルター。dt と時定数を使います。
function s=filterStep(u,h,T,s),s=s*T/(T+h)+u*h/(T+h);end

== matlab function Horizontal1804/FlightControl/TakeoffHoverControl/AttitudeControl/StickToAngleRate ==
  data: arg_arg_stick input single; arg_arg_angle output single; arg_branch input uint8; arg_arg_run input boolean; arg_arg_reset input boolean; arg_arg_lastRate input single; arg_arg_controlMode input single; arg_arg_directRate output single; arg_arg_resetError output single
function [arg_arg_angle,arg_arg_directRate,arg_arg_resetError]=stepFn(arg_arg_stick,arg_branch,arg_arg_run,arg_arg_reset,arg_arg_lastRate,arg_arg_controlMode)
% 概要：操縦スティックから角度・角速度目標を作ります。Stabilize は Roll/Pitch ±30°、Sport は非線形な角速度指令、Yaw は角速度指令です。低推力リセット時に中立値を記憶します。
%#codegen
% 1. 角度目標、スティック中立値、直前の指令を保持します。
persistent Angle Centers AngleCmd YawCmd;
if isempty(Angle),Angle=zeros(2,1,'single');Centers=zeros(3,1,'single');AngleCmd=zeros(2,1,'single');YawCmd=single(0);end
arg_arg_directRate=arg_arg_lastRate;arg_arg_resetError=Angle;
% 2. 通常飛行・着陸の分岐で操縦入力を更新し、モードに応じて角度または直接角速度を生成します。
commandCalled=arg_branch==2 || arg_branch==5;
if commandCalled
 if uint8(arg_arg_controlMode)==0 || arg_branch==5,AngleCmd=min(max(single(.4*double(arg_arg_stick(1:2))),single(-1)),single(1));end
 YawCmd=min(max(arg_arg_stick(3),single(-1)),single(1));
 arg_arg_directRate(3)=single(2*pi*double(YawCmd-Centers(3)));
 if uint8(arg_arg_controlMode)==1,arg_arg_directRate(1)=rateCommand(arg_arg_stick(1));arg_arg_directRate(2)=rateCommand(arg_arg_stick(2));end
end
% 3. リセット時の指令を中立値として保存します。
if arg_arg_reset,Centers(1:2)=AngleCmd;end
if arg_arg_reset,Centers(3)=YawCmd;end
% 4. Stabilize の角度目標を中立からの差分で作り、±30°に制限します。
if arg_arg_run && uint8(arg_arg_controlMode)==0
 limit=single(30*pi/180);Angle=min(max(single(.5*pi*double(AngleCmd-Centers(1:2))),-limit),limit);
end
% 5. 指定分岐とリセット条件を反映して公開する角速度を決めます。
if arg_branch==3,arg_arg_directRate(1)=single(0);end
if arg_arg_reset,arg_arg_directRate(:)=single(0);end
arg_arg_angle=Angle;
end
% 6. 局所関数：Sport の角速度カーブ。入力を ±1 に制限し、低入力の感度と最大 1600 deg/s の特性を維持します。
function y=rateCommand(x)
x=min(max(x,single(-1)),single(1));a=abs(x);t=a*(a*a*a*a*a*single(.5)+a*single(.5));
y=single(pi/180)*((single(1600)-single(70))*t+single(70)*a);if x<0,y=-y;end
end

== matlab function Horizontal1804/FlightControl/TakeoffHoverControl/AttitudeControl/SelectRateReference ==
  data: direct input single; rate output single; rollPID input single; pitchPID input single; angleEnable input boolean
function rate =stepFn(direct,rollPID,pitchPID,angleEnable)
% 概要：角速度 PID の目標 [Roll, Pitch, Yaw] を選びます。Stabilize で角度制御が有効なときだけ Roll/Pitch を角度 PID の出力へ置換し、Yaw と Sport の直接角速度目標はそのまま使います。
%#codegen
% 1. 直接角速度目標を初期値とし、角度ループが有効な軸だけを上書きします。
            rate=direct;if angleEnable,rate(1)=rollPID;rate(2)=pitchPID;end
end

== matlab function Horizontal1804/FlightControl/TakeoffHoverControl/FlightDiagnostics/ControlDiagnosticPack ==
  data: alt input single; diag output single; base input single; counter input uint16; zRef input single; thrust input single; angle input single; rate input single; rollTorque input single; pitchTorque input single; yawTorque input single; before input single
function diag =stepFn(alt,base,counter,zRef,thrust,angle,rate,rollTorque,pitchTorque,yawTorque,before)
% 概要：制御内部の観測値を 17 要素の single ベクトルにまとめます。ログの項目順は [高度制御状態; 基準推力; 離陸カウンター; 高度目標; 推力; 角度目標2; 角速度目標3; 軸補正3; 配分前モーター値4] です。制御判断は行いません。
%#codegen
% 1. 既存のログ順序を保って結合します。離陸カウンターだけを single へ変換します。
            diag=[alt;base;single(counter);zRef;thrust;angle;rate;rollTorque;pitchTorque;yawTorque;before];
end

== stateflow chart Horizontal1804/FlightControl/TakeoffHoverControl/FlightCommand/FinalizeFlightMode ==
  settings: description=Normal flight: finalize the mode; excessive acceleration and completed landing return to parking.
  state FinalModes [parallel]
    settings: executionOrder=1
    state OTHER
      en: mode=preMode;
    state INIT
      en: mode=uint8(0);
    state LANDING
      en: mode=uint8(5);
    state PARKING
      en: mode=uint8(3);
    state FLIGHT
      en: mode=uint8(2);
    state AVERAGE
      en: mode=uint8(1);
    (default) -> INIT
    (junction 27) -> OTHER [order 8]
    (junction 27) -> INIT [order 3] : [preMode==uint8(0)]
    FinalModes -> (junction 27) : decide
    (junction 27) -> AVERAGE [order 4] : [preMode==uint8(1)]
    (junction 27) -> LANDING [order 7] : [preMode==uint8(5)]
    (junction 27) -> FLIGHT [order 6] : [preMode==uint8(2)]
    (junction 27) -> PARKING [order 5] : [preMode==uint8(3)]
    (junction 27) -> PARKING [order 2] : [branch==5 && height<.1]
    (junction 27) -> PARKING [order 1] : [(branch==2 || branch==5) && overG==1]
  state CycleInput [parallel]
    en: mode=preMode;send(decide,FinalModes);
    du: mode=preMode;send(decide,FinalModes);
    settings: executionOrder=2
  note: Basic flight: takeoff, hover, landing and normal fault handling.
  data: branch input uint8; preMode input uint8; height input single; overG input uint8; mode output uint8
  events: decide local FUNCTION_CALL_EVENT
